simulink model "IEEE33_TR_TEMPORAL_RECOGNIZABILITY_MASTER"  (R2026b)
settings: Solver=ode23t  StopTime=0.2  MaxStep=1e-5
undefined symbols (not defined in the file): Three_PhaseBreaker_class, Three_PhaseSeriesRLCLoad_class, Three_PhaseSource_class, Three_PhaseV_IMeasuremen_class
libraries: ee_lib x146, nesl_utility x106, fl_lib x33, eeRmsMeasurement x2
(part 6 of 7)

== system IEEE33_TR_TEMPORAL_RECOGNIZABILITY_MASTER/Bus_3/CB3-1 ==
  com : Inport
  Add : Sum
  Circuit Breaker : ee_lib/Switches & Breakers/Circuit Breaker (Three-Phase)  port_option=ee.enum.threePhasePort.expanded  control_port_option=ee.enum.controlport.ps  R_closed=0.01 Ohm  G_open=Three_PhaseBreaker_class('open',1000000,Inf,[0.0166666666666667 0.0833333333333333],'on').objParamMappingDerived.NewDerivedParam.G_open 1/Ohm  threshold=0.5 V  breaker_behavior=ee.enum.switches.breakerBehavior.zeroCrossingEnable  i_th=1e-8 A
  Data Type Conversion : DataTypeConversion  OutDataTypeStr=double  SaturateOnIntegerOverflow=off  RndMeth=Floor
  NOT : Logic  Operator=NOT  IconShape=distinctive  AllPortsSameDT=off  OutDataTypeStr=boolean
  Simulink-PS Converter : nesl_utility/Simulink-PS Converter  PhysicalDomain=network_engine_domain  SubClassName=ps_input  LeftPortType=input  RightPortType=output  PseudoPeriodic=off  Frequencies=[]  NoiseDistribution=none  NoiseParameters=[]  Unit=1  AffineConversion=off  FilteringAndDerivatives=provide  SimscapeFilterOrder=1  InputFilterTimeConstant=0.001  UdotUserProvided=0
  Step : Step  Time=1e-6  InitialValue=Three_PhaseBreaker_class('open',1000000,Inf,[0.0166666666666667 0.0833333333333333],'on').objParamMappingDerived.NewDerivedParam.StepInitialValue  FinalValue=0  SampleTime=0
  A : PMIOPort  Side=Left
  B : PMIOPort  Port=2  Side=Left
  C : PMIOPort  Port=3  Side=Left
  a : PMIOPort  Port=4  Side=Right
  b : PMIOPort  Port=5  Side=Right
  c : PMIOPort  Port=6  Side=Right
  wires:
  com/1 -> Add/1
  Add/1 -> NOT/1
  Step/1 -> Add/2
  Data Type Conversion/1 -> Simulink-PS Converter/1
  NOT/1 -> Data Type Conversion/1
  connections:
  Circuit Breaker/LConn1 -- Simulink-PS Converter/RConn1
  c/RConn1 -- Circuit Breaker/RConn3
  b/RConn1 -- Circuit Breaker/RConn2
  a/RConn1 -- Circuit Breaker/RConn1
  Circuit Breaker/LConn4 -- C/RConn1
  Circuit Breaker/LConn3 -- B/RConn1
  Circuit Breaker/LConn2 -- A/RConn1

== system IEEE33_TR_TEMPORAL_RECOGNIZABILITY_MASTER/Bus_3/CB3-2 ==
  com : Inport
  Add : Sum
  Circuit Breaker : ee_lib/Switches & Breakers/Circuit Breaker (Three-Phase)  port_option=ee.enum.threePhasePort.expanded  control_port_option=ee.enum.controlport.ps  R_closed=0.01 Ohm  G_open=Three_PhaseBreaker_class('open',1000000,Inf,[0.0166666666666667 0.0833333333333333],'on').objParamMappingDerived.NewDerivedParam.G_open 1/Ohm  threshold=0.5 V  breaker_behavior=ee.enum.switches.breakerBehavior.zeroCrossingEnable  i_th=1e-8 A
  Data Type Conversion : DataTypeConversion  OutDataTypeStr=double  SaturateOnIntegerOverflow=off  RndMeth=Floor
  NOT : Logic  Operator=NOT  IconShape=distinctive  AllPortsSameDT=off  OutDataTypeStr=boolean
  Simulink-PS Converter : nesl_utility/Simulink-PS Converter  PhysicalDomain=network_engine_domain  SubClassName=ps_input  LeftPortType=input  RightPortType=output  PseudoPeriodic=off  Frequencies=[]  NoiseDistribution=none  NoiseParameters=[]  Unit=1  AffineConversion=off  FilteringAndDerivatives=provide  SimscapeFilterOrder=1  InputFilterTimeConstant=0.001  UdotUserProvided=0
  Step : Step  Time=1e-6  InitialValue=Three_PhaseBreaker_class('open',1000000,Inf,[0.0166666666666667 0.0833333333333333],'on').objParamMappingDerived.NewDerivedParam.StepInitialValue  FinalValue=0  SampleTime=0
  A : PMIOPort  Side=Left
  B : PMIOPort  Port=2  Side=Left
  C : PMIOPort  Port=3  Side=Left
  a : PMIOPort  Port=4  Side=Right
  b : PMIOPort  Port=5  Side=Right
  c : PMIOPort  Port=6  Side=Right
  wires:
  com/1 -> Add/1
  Add/1 -> NOT/1
  Step/1 -> Add/2
  Data Type Conversion/1 -> Simulink-PS Converter/1
  NOT/1 -> Data Type Conversion/1
  connections:
  Circuit Breaker/LConn1 -- Simulink-PS Converter/RConn1
  c/RConn1 -- Circuit Breaker/RConn3
  b/RConn1 -- Circuit Breaker/RConn2
  a/RConn1 -- Circuit Breaker/RConn1
  Circuit Breaker/LConn4 -- C/RConn1
  Circuit Breaker/LConn3 -- B/RConn1
  Circuit Breaker/LConn2 -- A/RConn1

== system IEEE33_TR_TEMPORAL_RECOGNIZABILITY_MASTER/Bus_3/VI Recorder6 ==
  Vrec : Inport
  Irec : Inport  Port=2
  tag scope: I2to3=global, V2to3=global
  wires:
  Vrec/1 -> [V2to3]
  Irec/1 -> [I2to3]

== system IEEE33_TR_TEMPORAL_RECOGNIZABILITY_MASTER/Bus_30/Bus Load 30 ==
  Electrical Reference : fl_lib/Electrical/Electrical Elements/Electrical Reference
  Wye-Connected Load : ee_lib/Passive/RLC Assemblies/Wye-Connected Load  port_option=ee.enum.threePhasePort.expanded  parameterization=2  component_structure=4  component_structure_PQ=4  R=1 Ohm  L=0.001 H  C=1e-6 F  VRated=11673.3176 V  FRated=60 Hz  P=200000 W  Qpos=600000 V*A  Qneg=Three_PhaseSeriesRLCLoad_class(0).objParamMappingDerived.NewDerivedParam.Qneg V*A  R_parasitic=1e-6 Ohm  G_parasitic=1e-6 1/Ohm  R_parasitic_PQ=1e-6 Ohm  G_parasitic_PQ=1e-6 1/Ohm  Vmag0=11673.3176 V  Vang0=0 deg  Freq0=60 Hz  IL_specify=on  IL_priority=High  IL=[ 0 0 0 ] A  IL_nominal_specify=off  IL_nominal_value=1  IL_nominal_unit=A  VC_specify=on  VC_priority=High  VC=[ 0 0 0 ] V  VC_nominal_specify=off  VC_nominal_value=1  VC_nominal_unit=V
  A : PMIOPort  Side=Left
  B : PMIOPort  Port=2  Side=Left
  C : PMIOPort  Port=3  Side=Left
  connections:
  Electrical Reference/LConn1 -- Wye-Connected Load/RConn1
  Wye-Connected Load/LConn3 -- C/RConn1
  Wye-Connected Load/LConn1 -- A/RConn1
  Wye-Connected Load/LConn2 -- B/RConn1

== system IEEE33_TR_TEMPORAL_RECOGNIZABILITY_MASTER/Bus_30/Bus_30 ==
  Current and Voltage Sensor (Three-Phase) : ee_lib/Sensors & Transducers/Current and Voltage Sensor (Three-Phase)  port_option=ee.enum.threePhasePort.expanded  vMeasurementType=1  outputUnit=2  SRated=100000000 V*A  VRated=500000 V  I_specify=off  I_priority=None  I=[ 0 0 0 ] A  I_nominal_specify=off  I_nominal_value=1  I_nominal_unit=A  V_specify=off  V_priority=None  V=[ 0 0 0 ] V  V_nominal_specify=off  V_nominal_value=1  V_nominal_unit=V
  Igain : Gain  Gain=Three_PhaseV_IMeasuremen_class('phase-to-phase','yes','off','off','off',100000000,500000).objParamMappingDerived.NewDerivedParam.IG
  PS-Simulink Converter : nesl_utility/PS-Simulink Converter  PhysicalDomain=network_engine_domain  SubClassName=ps_output  LeftPortType=input  RightPortType=output  PseudoPeriodic=off  Frequencies=[]  VectorFormat=1-D array  Unit=1  AffineConversion=off
  PS-Simulink Converter1 : nesl_utility/PS-Simulink Converter  PhysicalDomain=network_engine_domain  SubClassName=ps_output  LeftPortType=input  RightPortType=output  PseudoPeriodic=off  Frequencies=[]  VectorFormat=1-D array  Unit=1  AffineConversion=off
  Vgain : Gain  Gain=Three_PhaseV_IMeasuremen_class('phase-to-phase','yes','off','off','off',100000000,500000).objParamMappingDerived.NewDerivedParam.VG
  A : PMIOPort  Side=Left
  B : PMIOPort  Port=2  Side=Left
  C : PMIOPort  Port=3  Side=Left
  a : PMIOPort  Port=4  Side=Right
  b : PMIOPort  Port=5  Side=Right
  c : PMIOPort  Port=6  Side=Right
  Vabc : Outport  VectorParamsAs1DForOutWhenUnconnected=off
  Iabc : Outport  Port=2  VectorParamsAs1DForOutWhenUnconnected=off
  wires:
  Igain/1 -> Iabc/1
  Vgain/1 -> Vabc/1
  PS-Simulink Converter1/1 -> Igain/1
  PS-Simulink Converter/1 -> Vgain/1
  connections:
  Current and Voltage Sensor (Three-Phase)/RConn1 -- PS-Simulink Converter/LConn1
  Current and Voltage Sensor (Three-Phase)/RConn2 -- PS-Simulink Converter1/LConn1
  Current and Voltage Sensor (Three-Phase)/RConn5 -- c/RConn1
  Current and Voltage Sensor (Three-Phase)/RConn4 -- b/RConn1
  Current and Voltage Sensor (Three-Phase)/RConn3 -- a/RConn1
  Current and Voltage Sensor (Three-Phase)/LConn3 -- C/RConn1
  Current and Voltage Sensor (Three-Phase)/LConn1 -- A/RConn1
  Current and Voltage Sensor (Three-Phase)/LConn2 -- B/RConn1

== system IEEE33_TR_TEMPORAL_RECOGNIZABILITY_MASTER/Bus_30/CB3-2 ==
  com : Inport
  Add : Sum
  Circuit Breaker : ee_lib/Switches & Breakers/Circuit Breaker (Three-Phase)  port_option=ee.enum.threePhasePort.expanded  control_port_option=ee.enum.controlport.ps  R_closed=0.01 Ohm  G_open=Three_PhaseBreaker_class('open',1000000,Inf,[0.0166666666666667 0.0833333333333333],'on').objParamMappingDerived.NewDerivedParam.G_open 1/Ohm  threshold=0.5 V  breaker_behavior=ee.enum.switches.breakerBehavior.zeroCrossingEnable  i_th=1e-8 A
  Data Type Conversion : DataTypeConversion  OutDataTypeStr=double  SaturateOnIntegerOverflow=off  RndMeth=Floor
  NOT : Logic  Operator=NOT  IconShape=distinctive  AllPortsSameDT=off  OutDataTypeStr=boolean
  Simulink-PS Converter : nesl_utility/Simulink-PS Converter  PhysicalDomain=network_engine_domain  SubClassName=ps_input  LeftPortType=input  RightPortType=output  PseudoPeriodic=off  Frequencies=[]  NoiseDistribution=none  NoiseParameters=[]  Unit=1  AffineConversion=off  FilteringAndDerivatives=provide  SimscapeFilterOrder=1  InputFilterTimeConstant=0.001  UdotUserProvided=0
  Step : Step  Time=1e-6  InitialValue=Three_PhaseBreaker_class('open',1000000,Inf,[0.0166666666666667 0.0833333333333333],'on').objParamMappingDerived.NewDerivedParam.StepInitialValue  FinalValue=0  SampleTime=0
  A : PMIOPort  Side=Left
  B : PMIOPort  Port=2  Side=Left
  C : PMIOPort  Port=3  Side=Left
  a : PMIOPort  Port=4  Side=Right
  b : PMIOPort  Port=5  Side=Right
  c : PMIOPort  Port=6  Side=Right
  wires:
  com/1 -> Add/1
  Add/1 -> NOT/1
  Step/1 -> Add/2
  Data Type Conversion/1 -> Simulink-PS Converter/1
  NOT/1 -> Data Type Conversion/1
  connections:
  Circuit Breaker/LConn1 -- Simulink-PS Converter/RConn1
  c/RConn1 -- Circuit Breaker/RConn3
  b/RConn1 -- Circuit Breaker/RConn2
  a/RConn1 -- Circuit Breaker/RConn1
  Circuit Breaker/LConn4 -- C/RConn1
  Circuit Breaker/LConn3 -- B/RConn1
  Circuit Breaker/LConn2 -- A/RConn1

== system IEEE33_TR_TEMPORAL_RECOGNIZABILITY_MASTER/Bus_30/VI Recorder26 ==
  Vrec : Inport
  Irec : Inport  Port=2
  tag scope: I29to30=global, V29to30=global
  wires:
  Vrec/1 -> [V29to30]
  Irec/1 -> [I29to30]

== system IEEE33_TR_TEMPORAL_RECOGNIZABILITY_MASTER/Bus_31/Bus Load 31 ==
  Electrical Reference : fl_lib/Electrical/Electrical Elements/Electrical Reference
  Wye-Connected Load : ee_lib/Passive/RLC Assemblies/Wye-Connected Load  port_option=ee.enum.threePhasePort.expanded  parameterization=2  component_structure=4  component_structure_PQ=4  R=1 Ohm  L=0.001 H  C=1e-6 F  VRated=11620.7279 V  FRated=60 Hz  P=150000 W  Qpos=70000 V*A  Qneg=Three_PhaseSeriesRLCLoad_class(0).objParamMappingDerived.NewDerivedParam.Qneg V*A  R_parasitic=1e-6 Ohm  G_parasitic=1e-6 1/Ohm  R_parasitic_PQ=1e-6 Ohm  G_parasitic_PQ=1e-6 1/Ohm  Vmag0=11620.7279 V  Vang0=0 deg  Freq0=60 Hz  IL_specify=on  IL_priority=High  IL=[ 0 0 0 ] A  IL_nominal_specify=off  IL_nominal_value=1  IL_nominal_unit=A  VC_specify=on  VC_priority=High  VC=[ 0 0 0 ] V  VC_nominal_specify=off  VC_nominal_value=1  VC_nominal_unit=V
  A : PMIOPort  Side=Left
  B : PMIOPort  Port=2  Side=Left
  C : PMIOPort  Port=3  Side=Left
  connections:
  Electrical Reference/LConn1 -- Wye-Connected Load/RConn1
  Wye-Connected Load/LConn3 -- C/RConn1
  Wye-Connected Load/LConn1 -- A/RConn1
  Wye-Connected Load/LConn2 -- B/RConn1

== system IEEE33_TR_TEMPORAL_RECOGNIZABILITY_MASTER/Bus_31/Bus_31 ==
  Current and Voltage Sensor (Three-Phase) : ee_lib/Sensors & Transducers/Current and Voltage Sensor (Three-Phase)  port_option=ee.enum.threePhasePort.expanded  vMeasurementType=1  outputUnit=2  SRated=100000000 V*A  VRated=500000 V  I_specify=off  I_priority=None  I=[ 0 0 0 ] A  I_nominal_specify=off  I_nominal_value=1  I_nominal_unit=A  V_specify=off  V_priority=None  V=[ 0 0 0 ] V  V_nominal_specify=off  V_nominal_value=1  V_nominal_unit=V
  Igain : Gain  Gain=Three_PhaseV_IMeasuremen_class('phase-to-phase','yes','off','off','off',100000000,500000).objParamMappingDerived.NewDerivedParam.IG
  PS-Simulink Converter : nesl_utility/PS-Simulink Converter  PhysicalDomain=network_engine_domain  SubClassName=ps_output  LeftPortType=input  RightPortType=output  PseudoPeriodic=off  Frequencies=[]  VectorFormat=1-D array  Unit=1  AffineConversion=off
  PS-Simulink Converter1 : nesl_utility/PS-Simulink Converter  PhysicalDomain=network_engine_domain  SubClassName=ps_output  LeftPortType=input  RightPortType=output  PseudoPeriodic=off  Frequencies=[]  VectorFormat=1-D array  Unit=1  AffineConversion=off
  Vgain : Gain  Gain=Three_PhaseV_IMeasuremen_class('phase-to-phase','yes','off','off','off',100000000,500000).objParamMappingDerived.NewDerivedParam.VG
  A : PMIOPort  Side=Left
  B : PMIOPort  Port=2  Side=Left
  C : PMIOPort  Port=3  Side=Left
  a : PMIOPort  Port=4  Side=Right
  b : PMIOPort  Port=5  Side=Right
  c : PMIOPort  Port=6  Side=Right
  Vabc : Outport  VectorParamsAs1DForOutWhenUnconnected=off
  Iabc : Outport  Port=2  VectorParamsAs1DForOutWhenUnconnected=off
  wires:
  Igain/1 -> Iabc/1
  Vgain/1 -> Vabc/1
  PS-Simulink Converter1/1 -> Igain/1
  PS-Simulink Converter/1 -> Vgain/1
  connections:
  Current and Voltage Sensor (Three-Phase)/RConn1 -- PS-Simulink Converter/LConn1
  Current and Voltage Sensor (Three-Phase)/RConn2 -- PS-Simulink Converter1/LConn1
  Current and Voltage Sensor (Three-Phase)/RConn5 -- c/RConn1
  Current and Voltage Sensor (Three-Phase)/RConn4 -- b/RConn1
  Current and Voltage Sensor (Three-Phase)/RConn3 -- a/RConn1
  Current and Voltage Sensor (Three-Phase)/LConn3 -- C/RConn1
  Current and Voltage Sensor (Three-Phase)/LConn1 -- A/RConn1
  Current and Voltage Sensor (Three-Phase)/LConn2 -- B/RConn1

== system IEEE33_TR_TEMPORAL_RECOGNIZABILITY_MASTER/Bus_31/CB3-2 ==
  com : Inport
  Add : Sum
  Circuit Breaker : ee_lib/Switches & Breakers/Circuit Breaker (Three-Phase)  port_option=ee.enum.threePhasePort.expanded  control_port_option=ee.enum.controlport.ps  R_closed=0.01 Ohm  G_open=Three_PhaseBreaker_class('open',1000000,Inf,[0.0166666666666667 0.0833333333333333],'on').objParamMappingDerived.NewDerivedParam.G_open 1/Ohm  threshold=0.5 V  breaker_behavior=ee.enum.switches.breakerBehavior.zeroCrossingEnable  i_th=1e-8 A
  Data Type Conversion : DataTypeConversion  OutDataTypeStr=double  SaturateOnIntegerOverflow=off  RndMeth=Floor
  NOT : Logic  Operator=NOT  IconShape=distinctive  AllPortsSameDT=off  OutDataTypeStr=boolean
  Simulink-PS Converter : nesl_utility/Simulink-PS Converter  PhysicalDomain=network_engine_domain  SubClassName=ps_input  LeftPortType=input  RightPortType=output  PseudoPeriodic=off  Frequencies=[]  NoiseDistribution=none  NoiseParameters=[]  Unit=1  AffineConversion=off  FilteringAndDerivatives=provide  SimscapeFilterOrder=1  InputFilterTimeConstant=0.001  UdotUserProvided=0
  Step : Step  Time=1e-6  InitialValue=Three_PhaseBreaker_class('open',1000000,Inf,[0.0166666666666667 0.0833333333333333],'on').objParamMappingDerived.NewDerivedParam.StepInitialValue  FinalValue=0  SampleTime=0
  A : PMIOPort  Side=Left
  B : PMIOPort  Port=2  Side=Left
  C : PMIOPort  Port=3  Side=Left
  a : PMIOPort  Port=4  Side=Right
  b : PMIOPort  Port=5  Side=Right
  c : PMIOPort  Port=6  Side=Right
  wires:
  com/1 -> Add/1
  Add/1 -> NOT/1
  Step/1 -> Add/2
  Data Type Conversion/1 -> Simulink-PS Converter/1
  NOT/1 -> Data Type Conversion/1
  connections:
  Circuit Breaker/LConn1 -- Simulink-PS Converter/RConn1
  c/RConn1 -- Circuit Breaker/RConn3
  b/RConn1 -- Circuit Breaker/RConn2
  a/RConn1 -- Circuit Breaker/RConn1
  Circuit Breaker/LConn4 -- C/RConn1
  Circuit Breaker/LConn3 -- B/RConn1
  Circuit Breaker/LConn2 -- A/RConn1

== system IEEE33_TR_TEMPORAL_RECOGNIZABILITY_MASTER/Bus_31/VI Recorder27 ==
  Vrec : Inport
  Irec : Inport  Port=2
  tag scope: I30to31=global, V30to31=global
  wires:
  Vrec/1 -> [V30to31]
  Irec/1 -> [I30to31]

== system IEEE33_TR_TEMPORAL_RECOGNIZABILITY_MASTER/Bus_32/Bus Load 32 ==
  Electrical Reference : fl_lib/Electrical/Electrical Elements/Electrical Reference
  Wye-Connected Load : ee_lib/Passive/RLC Assemblies/Wye-Connected Load  port_option=ee.enum.threePhasePort.expanded  parameterization=2  component_structure=4  component_structure_PQ=4  R=1 Ohm  L=0.001 H  C=1e-6 F  VRated=11609.1567 V  FRated=60 Hz  P=210000 W  Qpos=100000 V*A  Qneg=Three_PhaseSeriesRLCLoad_class(0).objParamMappingDerived.NewDerivedParam.Qneg V*A  R_parasitic=1e-6 Ohm  G_parasitic=1e-6 1/Ohm  R_parasitic_PQ=1e-6 Ohm  G_parasitic_PQ=1e-6 1/Ohm  Vmag0=11609.1567 V  Vang0=0 deg  Freq0=60 Hz  IL_specify=on  IL_priority=High  IL=[ 0 0 0 ] A  IL_nominal_specify=off  IL_nominal_value=1  IL_nominal_unit=A  VC_specify=on  VC_priority=High  VC=[ 0 0 0 ] V  VC_nominal_specify=off  VC_nominal_value=1  VC_nominal_unit=V
  A : PMIOPort  Side=Left
  B : PMIOPort  Port=2  Side=Left
  C : PMIOPort  Port=3  Side=Left
  connections:
  Electrical Reference/LConn1 -- Wye-Connected Load/RConn1
  Wye-Connected Load/LConn3 -- C/RConn1
  Wye-Connected Load/LConn1 -- A/RConn1
  Wye-Connected Load/LConn2 -- B/RConn1

== system IEEE33_TR_TEMPORAL_RECOGNIZABILITY_MASTER/Bus_32/Bus_32 ==
  Current and Voltage Sensor (Three-Phase) : ee_lib/Sensors & Transducers/Current and Voltage Sensor (Three-Phase)  port_option=ee.enum.threePhasePort.expanded  vMeasurementType=1  outputUnit=2  SRated=100000000 V*A  VRated=500000 V  I_specify=off  I_priority=None  I=[ 0 0 0 ] A  I_nominal_specify=off  I_nominal_value=1  I_nominal_unit=A  V_specify=off  V_priority=None  V=[ 0 0 0 ] V  V_nominal_specify=off  V_nominal_value=1  V_nominal_unit=V
  Igain : Gain  Gain=Three_PhaseV_IMeasuremen_class('phase-to-phase','yes','off','off','off',100000000,500000).objParamMappingDerived.NewDerivedParam.IG
  PS-Simulink Converter : nesl_utility/PS-Simulink Converter  PhysicalDomain=network_engine_domain  SubClassName=ps_output  LeftPortType=input  RightPortType=output  PseudoPeriodic=off  Frequencies=[]  VectorFormat=1-D array  Unit=1  AffineConversion=off
  PS-Simulink Converter1 : nesl_utility/PS-Simulink Converter  PhysicalDomain=network_engine_domain  SubClassName=ps_output  LeftPortType=input  RightPortType=output  PseudoPeriodic=off  Frequencies=[]  VectorFormat=1-D array  Unit=1  AffineConversion=off
  Vgain : Gain  Gain=Three_PhaseV_IMeasuremen_class('phase-to-phase','yes','off','off','off',100000000,500000).objParamMappingDerived.NewDerivedParam.VG
  A : PMIOPort  Side=Left
  B : PMIOPort  Port=2  Side=Left
  C : PMIOPort  Port=3  Side=Left
  a : PMIOPort  Port=4  Side=Right
  b : PMIOPort  Port=5  Side=Right
  c : PMIOPort  Port=6  Side=Right
  Vabc : Outport  VectorParamsAs1DForOutWhenUnconnected=off
  Iabc : Outport  Port=2  VectorParamsAs1DForOutWhenUnconnected=off
  wires:
  Igain/1 -> Iabc/1
  Vgain/1 -> Vabc/1
  PS-Simulink Converter1/1 -> Igain/1
  PS-Simulink Converter/1 -> Vgain/1
  connections:
  Current and Voltage Sensor (Three-Phase)/RConn1 -- PS-Simulink Converter/LConn1
  Current and Voltage Sensor (Three-Phase)/RConn2 -- PS-Simulink Converter1/LConn1
  Current and Voltage Sensor (Three-Phase)/RConn5 -- c/RConn1
  Current and Voltage Sensor (Three-Phase)/RConn4 -- b/RConn1
  Current and Voltage Sensor (Three-Phase)/RConn3 -- a/RConn1
  Current and Voltage Sensor (Three-Phase)/LConn3 -- C/RConn1
  Current and Voltage Sensor (Three-Phase)/LConn1 -- A/RConn1
  Current and Voltage Sensor (Three-Phase)/LConn2 -- B/RConn1

== system IEEE33_TR_TEMPORAL_RECOGNIZABILITY_MASTER/Bus_32/CB3-2 ==
  com : Inport
  Add : Sum
  Circuit Breaker : ee_lib/Switches & Breakers/Circuit Breaker (Three-Phase)  port_option=ee.enum.threePhasePort.expanded  control_port_option=ee.enum.controlport.ps  R_closed=0.01 Ohm  G_open=Three_PhaseBreaker_class('open',1000000,Inf,[0.0166666666666667 0.0833333333333333],'on').objParamMappingDerived.NewDerivedParam.G_open 1/Ohm  threshold=0.5 V  breaker_behavior=ee.enum.switches.breakerBehavior.zeroCrossingEnable  i_th=1e-8 A
  Data Type Conversion : DataTypeConversion  OutDataTypeStr=double  SaturateOnIntegerOverflow=off  RndMeth=Floor
  NOT : Logic  Operator=NOT  IconShape=distinctive  AllPortsSameDT=off  OutDataTypeStr=boolean
  Simulink-PS Converter : nesl_utility/Simulink-PS Converter  PhysicalDomain=network_engine_domain  SubClassName=ps_input  LeftPortType=input  RightPortType=output  PseudoPeriodic=off  Frequencies=[]  NoiseDistribution=none  NoiseParameters=[]  Unit=1  AffineConversion=off  FilteringAndDerivatives=provide  SimscapeFilterOrder=1  InputFilterTimeConstant=0.001  UdotUserProvided=0
  Step : Step  Time=1e-6  InitialValue=Three_PhaseBreaker_class('open',1000000,Inf,[0.0166666666666667 0.0833333333333333],'on').objParamMappingDerived.NewDerivedParam.StepInitialValue  FinalValue=0  SampleTime=0
  A : PMIOPort  Side=Left
  B : PMIOPort  Port=2  Side=Left
  C : PMIOPort  Port=3  Side=Left
  a : PMIOPort  Port=4  Side=Right
  b : PMIOPort  Port=5  Side=Right
  c : PMIOPort  Port=6  Side=Right
  wires:
  com/1 -> Add/1
  Add/1 -> NOT/1
  Step/1 -> Add/2
  Data Type Conversion/1 -> Simulink-PS Converter/1
  NOT/1 -> Data Type Conversion/1
  connections:
  Circuit Breaker/LConn1 -- Simulink-PS Converter/RConn1
  c/RConn1 -- Circuit Breaker/RConn3
  b/RConn1 -- Circuit Breaker/RConn2
  a/RConn1 -- Circuit Breaker/RConn1
  Circuit Breaker/LConn4 -- C/RConn1
  Circuit Breaker/LConn3 -- B/RConn1
  Circuit Breaker/LConn2 -- A/RConn1

== system IEEE33_TR_TEMPORAL_RECOGNIZABILITY_MASTER/Bus_32/VI Recorder28 ==
  Vrec : Inport
  Irec : Inport  Port=2
  tag scope: I31to32=global, V31to32=global
  wires:
  Vrec/1 -> [V31to32]
  Irec/1 -> [I31to32]

== system IEEE33_TR_TEMPORAL_RECOGNIZABILITY_MASTER/Bus_33/Bus Load 33 ==
  Electrical Reference : fl_lib/Electrical/Electrical Elements/Electrical Reference
  Wye-Connected Load : ee_lib/Passive/RLC Assemblies/Wye-Connected Load  port_option=ee.enum.threePhasePort.expanded  parameterization=2  component_structure=4  component_structure_PQ=4  R=1 Ohm  L=0.001 H  C=1e-6 F  VRated=11605.5739 V  FRated=60 Hz  P=60000 W  Qpos=40000 V*A  Qneg=Three_PhaseSeriesRLCLoad_class(0).objParamMappingDerived.NewDerivedParam.Qneg V*A  R_parasitic=1e-6 Ohm  G_parasitic=1e-6 1/Ohm  R_parasitic_PQ=1e-6 Ohm  G_parasitic_PQ=1e-6 1/Ohm  Vmag0=11605.5739 V  Vang0=0 deg  Freq0=60 Hz  IL_specify=on  IL_priority=High  IL=[ 0 0 0 ] A  IL_nominal_specify=off  IL_nominal_value=1  IL_nominal_unit=A  VC_specify=on  VC_priority=High  VC=[ 0 0 0 ] V  VC_nominal_specify=off  VC_nominal_value=1  VC_nominal_unit=V
  A : PMIOPort  Side=Left
  B : PMIOPort  Port=2  Side=Left
  C : PMIOPort  Port=3  Side=Left
  connections:
  Electrical Reference/LConn1 -- Wye-Connected Load/RConn1
  Wye-Connected Load/LConn3 -- C/RConn1
  Wye-Connected Load/LConn1 -- A/RConn1
  Wye-Connected Load/LConn2 -- B/RConn1

== system IEEE33_TR_TEMPORAL_RECOGNIZABILITY_MASTER/Bus_33/Bus_33 ==
  Current and Voltage Sensor (Three-Phase) : ee_lib/Sensors & Transducers/Current and Voltage Sensor (Three-Phase)  port_option=ee.enum.threePhasePort.expanded  vMeasurementType=1  outputUnit=2  SRated=100000000 V*A  VRated=500000 V  I_specify=off  I_priority=None  I=[ 0 0 0 ] A  I_nominal_specify=off  I_nominal_value=1  I_nominal_unit=A  V_specify=off  V_priority=None  V=[ 0 0 0 ] V  V_nominal_specify=off  V_nominal_value=1  V_nominal_unit=V
  Igain : Gain  Gain=Three_PhaseV_IMeasuremen_class('phase-to-phase','yes','off','off','off',100000000,500000).objParamMappingDerived.NewDerivedParam.IG
  PS-Simulink Converter : nesl_utility/PS-Simulink Converter  PhysicalDomain=network_engine_domain  SubClassName=ps_output  LeftPortType=input  RightPortType=output  PseudoPeriodic=off  Frequencies=[]  VectorFormat=1-D array  Unit=1  AffineConversion=off
  PS-Simulink Converter1 : nesl_utility/PS-Simulink Converter  PhysicalDomain=network_engine_domain  SubClassName=ps_output  LeftPortType=input  RightPortType=output  PseudoPeriodic=off  Frequencies=[]  VectorFormat=1-D array  Unit=1  AffineConversion=off
  Vgain : Gain  Gain=Three_PhaseV_IMeasuremen_class('phase-to-phase','yes','off','off','off',100000000,500000).objParamMappingDerived.NewDerivedParam.VG
  A : PMIOPort  Side=Left
  B : PMIOPort  Port=2  Side=Left
  C : PMIOPort  Port=3  Side=Left
  a : PMIOPort  Port=4  Side=Right
  b : PMIOPort  Port=5  Side=Right
  c : PMIOPort  Port=6  Side=Right
  Vabc : Outport  VectorParamsAs1DForOutWhenUnconnected=off
  Iabc : Outport  Port=2  VectorParamsAs1DForOutWhenUnconnected=off
  wires:
  Igain/1 -> Iabc/1
  Vgain/1 -> Vabc/1
  PS-Simulink Converter1/1 -> Igain/1
  PS-Simulink Converter/1 -> Vgain/1
  connections:
  Current and Voltage Sensor (Three-Phase)/RConn1 -- PS-Simulink Converter/LConn1
  Current and Voltage Sensor (Three-Phase)/RConn2 -- PS-Simulink Converter1/LConn1
  Current and Voltage Sensor (Three-Phase)/RConn5 -- c/RConn1
  Current and Voltage Sensor (Three-Phase)/RConn4 -- b/RConn1
  Current and Voltage Sensor (Three-Phase)/RConn3 -- a/RConn1
  Current and Voltage Sensor (Three-Phase)/LConn3 -- C/RConn1
  Current and Voltage Sensor (Three-Phase)/LConn1 -- A/RConn1
  Current and Voltage Sensor (Three-Phase)/LConn2 -- B/RConn1

== system IEEE33_TR_TEMPORAL_RECOGNIZABILITY_MASTER/Bus_33/VI Recorder29 ==
  Vrec : Inport
  Irec : Inport  Port=2
  tag scope: I32to33=global, V32to33=global
  wires:
  Vrec/1 -> [V32to33]
  Irec/1 -> [I32to33]

== system IEEE33_TR_TEMPORAL_RECOGNIZABILITY_MASTER/Bus_4/Bus Load 4 ==
  Electrical Reference : fl_lib/Electrical/Electrical Elements/Electrical Reference
  Wye-Connected Load : ee_lib/Passive/RLC Assemblies/Wye-Connected Load  port_option=ee.enum.threePhasePort.expanded  parameterization=2  component_structure=4  component_structure_PQ=4  R=1 Ohm  L=0.001 H  C=1e-6 F  VRated=12349.6274 V  FRated=60 Hz  P=120000 W  Qpos=80000 V*A  Qneg=Three_PhaseSeriesRLCLoad_class(0).objParamMappingDerived.NewDerivedParam.Qneg V*A  R_parasitic=1e-6 Ohm  G_parasitic=1e-6 1/Ohm  R_parasitic_PQ=1e-6 Ohm  G_parasitic_PQ=1e-6 1/Ohm  Vmag0=12349.6274 V  Vang0=0 deg  Freq0=60 Hz  IL_specify=on  IL_priority=High  IL=[ 0 0 0 ] A  IL_nominal_specify=off  IL_nominal_value=1  IL_nominal_unit=A  VC_specify=on  VC_priority=High  VC=[ 0 0 0 ] V  VC_nominal_specify=off  VC_nominal_value=1  VC_nominal_unit=V
  A : PMIOPort  Side=Left
  B : PMIOPort  Port=2  Side=Left
  C : PMIOPort  Port=3  Side=Left
  connections:
  Electrical Reference/LConn1 -- Wye-Connected Load/RConn1
  Wye-Connected Load/LConn3 -- C/RConn1
  Wye-Connected Load/LConn1 -- A/RConn1
  Wye-Connected Load/LConn2 -- B/RConn1

== system IEEE33_TR_TEMPORAL_RECOGNIZABILITY_MASTER/Bus_4/Bus_4 ==
  Current and Voltage Sensor (Three-Phase) : ee_lib/Sensors & Transducers/Current and Voltage Sensor (Three-Phase)  port_option=ee.enum.threePhasePort.expanded  vMeasurementType=1  outputUnit=2  SRated=100000000 V*A  VRated=500000 V  I_specify=off  I_priority=None  I=[ 0 0 0 ] A  I_nominal_specify=off  I_nominal_value=1  I_nominal_unit=A  V_specify=off  V_priority=None  V=[ 0 0 0 ] V  V_nominal_specify=off  V_nominal_value=1  V_nominal_unit=V
  Igain : Gain  Gain=Three_PhaseV_IMeasuremen_class('phase-to-phase','yes','off','off','off',100000000,500000).objParamMappingDerived.NewDerivedParam.IG
  PS-Simulink Converter : nesl_utility/PS-Simulink Converter  PhysicalDomain=network_engine_domain  SubClassName=ps_output  LeftPortType=input  RightPortType=output  PseudoPeriodic=off  Frequencies=[]  VectorFormat=1-D array  Unit=1  AffineConversion=off
  PS-Simulink Converter1 : nesl_utility/PS-Simulink Converter  PhysicalDomain=network_engine_domain  SubClassName=ps_output  LeftPortType=input  RightPortType=output  PseudoPeriodic=off  Frequencies=[]  VectorFormat=1-D array  Unit=1  AffineConversion=off
  Vgain : Gain  Gain=Three_PhaseV_IMeasuremen_class('phase-to-phase','yes','off','off','off',100000000,500000).objParamMappingDerived.NewDerivedParam.VG
  A : PMIOPort  Side=Left
  B : PMIOPort  Port=2  Side=Left
  C : PMIOPort  Port=3  Side=Left
  a : PMIOPort  Port=4  Side=Right
  b : PMIOPort  Port=5  Side=Right
  c : PMIOPort  Port=6  Side=Right
  Vabc : Outport  VectorParamsAs1DForOutWhenUnconnected=off
  Iabc : Outport  Port=2  VectorParamsAs1DForOutWhenUnconnected=off
  wires:
  Igain/1 -> Iabc/1
  Vgain/1 -> Vabc/1
  PS-Simulink Converter1/1 -> Igain/1
  PS-Simulink Converter/1 -> Vgain/1
  connections:
  Current and Voltage Sensor (Three-Phase)/RConn1 -- PS-Simulink Converter/LConn1
  Current and Voltage Sensor (Three-Phase)/RConn2 -- PS-Simulink Converter1/LConn1
  Current and Voltage Sensor (Three-Phase)/RConn5 -- c/RConn1
  Current and Voltage Sensor (Three-Phase)/RConn4 -- b/RConn1
  Current and Voltage Sensor (Three-Phase)/RConn3 -- a/RConn1
  Current and Voltage Sensor (Three-Phase)/LConn3 -- C/RConn1
  Current and Voltage Sensor (Three-Phase)/LConn1 -- A/RConn1
  Current and Voltage Sensor (Three-Phase)/LConn2 -- B/RConn1

== system IEEE33_TR_TEMPORAL_RECOGNIZABILITY_MASTER/Bus_4/CB3-2 ==
  com : Inport
  Add : Sum
  Circuit Breaker : ee_lib/Switches & Breakers/Circuit Breaker (Three-Phase)  port_option=ee.enum.threePhasePort.expanded  control_port_option=ee.enum.controlport.ps  R_closed=0.01 Ohm  G_open=Three_PhaseBreaker_class('open',1000000,Inf,[0.0166666666666667 0.0833333333333333],'on').objParamMappingDerived.NewDerivedParam.G_open 1/Ohm  threshold=0.5 V  breaker_behavior=ee.enum.switches.breakerBehavior.zeroCrossingEnable  i_th=1e-8 A
  Data Type Conversion : DataTypeConversion  OutDataTypeStr=double  SaturateOnIntegerOverflow=off  RndMeth=Floor
  NOT : Logic  Operator=NOT  IconShape=distinctive  AllPortsSameDT=off  OutDataTypeStr=boolean
  Simulink-PS Converter : nesl_utility/Simulink-PS Converter  PhysicalDomain=network_engine_domain  SubClassName=ps_input  LeftPortType=input  RightPortType=output  PseudoPeriodic=off  Frequencies=[]  NoiseDistribution=none  NoiseParameters=[]  Unit=1  AffineConversion=off  FilteringAndDerivatives=provide  SimscapeFilterOrder=1  InputFilterTimeConstant=0.001  UdotUserProvided=0
  Step : Step  Time=1e-6  InitialValue=Three_PhaseBreaker_class('open',1000000,Inf,[0.0166666666666667 0.0833333333333333],'on').objParamMappingDerived.NewDerivedParam.StepInitialValue  FinalValue=0  SampleTime=0
  A : PMIOPort  Side=Left
  B : PMIOPort  Port=2  Side=Left
  C : PMIOPort  Port=3  Side=Left
  a : PMIOPort  Port=4  Side=Right
  b : PMIOPort  Port=5  Side=Right
  c : PMIOPort  Port=6  Side=Right
  wires:
  com/1 -> Add/1
  Add/1 -> NOT/1
  Step/1 -> Add/2
  Data Type Conversion/1 -> Simulink-PS Converter/1
  NOT/1 -> Data Type Conversion/1
  connections:
  Circuit Breaker/LConn1 -- Simulink-PS Converter/RConn1
  c/RConn1 -- Circuit Breaker/RConn3
  b/RConn1 -- Circuit Breaker/RConn2
  a/RConn1 -- Circuit Breaker/RConn1
  Circuit Breaker/LConn4 -- C/RConn1
  Circuit Breaker/LConn3 -- B/RConn1
  Circuit Breaker/LConn2 -- A/RConn1

== system IEEE33_TR_TEMPORAL_RECOGNIZABILITY_MASTER/Bus_4/VI Recorder7 ==
  Vrec : Inport
  Irec : Inport  Port=2
  tag scope: I3to4=global, V3to4=global
  wires:
  Vrec/1 -> [V3to4]
  Irec/1 -> [I3to4]

== system IEEE33_TR_TEMPORAL_RECOGNIZABILITY_MASTER/Bus_5/Bus Load 5 ==
  Electrical Reference : fl_lib/Electrical/Electrical Elements/Electrical Reference
  Wye-Connected Load : ee_lib/Passive/RLC Assemblies/Wye-Connected Load  port_option=ee.enum.threePhasePort.expanded  parameterization=2  component_structure=4  component_structure_PQ=4  R=1 Ohm  L=0.001 H  C=1e-6 F  VRated=12256.1207 V  FRated=60 Hz  P=60000 W  Qpos=30000 V*A  Qneg=Three_PhaseSeriesRLCLoad_class(0).objParamMappingDerived.NewDerivedParam.Qneg V*A  R_parasitic=1e-6 Ohm  G_parasitic=1e-6 1/Ohm  R_parasitic_PQ=1e-6 Ohm  G_parasitic_PQ=1e-6 1/Ohm  Vmag0=12256.1207 V  Vang0=0 deg  Freq0=60 Hz  IL_specify=on  IL_priority=High  IL=[ 0 0 0 ] A  IL_nominal_specify=off  IL_nominal_value=1  IL_nominal_unit=A  VC_specify=on  VC_priority=High  VC=[ 0 0 0 ] V  VC_nominal_specify=off  VC_nominal_value=1  VC_nominal_unit=V
  A : PMIOPort  Side=Left
  B : PMIOPort  Port=2  Side=Left
  C : PMIOPort  Port=3  Side=Left
  connections:
  Electrical Reference/LConn1 -- Wye-Connected Load/RConn1
  Wye-Connected Load/LConn3 -- C/RConn1
  Wye-Connected Load/LConn1 -- A/RConn1
  Wye-Connected Load/LConn2 -- B/RConn1

== system IEEE33_TR_TEMPORAL_RECOGNIZABILITY_MASTER/Bus_5/Bus_5 ==
  Current and Voltage Sensor (Three-Phase) : ee_lib/Sensors & Transducers/Current and Voltage Sensor (Three-Phase)  port_option=ee.enum.threePhasePort.expanded  vMeasurementType=1  outputUnit=2  SRated=100000000 V*A  VRated=500000 V  I_specify=off  I_priority=None  I=[ 0 0 0 ] A  I_nominal_specify=off  I_nominal_value=1  I_nominal_unit=A  V_specify=off  V_priority=None  V=[ 0 0 0 ] V  V_nominal_specify=off  V_nominal_value=1  V_nominal_unit=V
  Igain : Gain  Gain=Three_PhaseV_IMeasuremen_class('phase-to-phase','yes','off','off','off',100000000,500000).objParamMappingDerived.NewDerivedParam.IG
  PS-Simulink Converter : nesl_utility/PS-Simulink Converter  PhysicalDomain=network_engine_domain  SubClassName=ps_output  LeftPortType=input  RightPortType=output  PseudoPeriodic=off  Frequencies=[]  VectorFormat=1-D array  Unit=1  AffineConversion=off
  PS-Simulink Converter1 : nesl_utility/PS-Simulink Converter  PhysicalDomain=network_engine_domain  SubClassName=ps_output  LeftPortType=input  RightPortType=output  PseudoPeriodic=off  Frequencies=[]  VectorFormat=1-D array  Unit=1  AffineConversion=off
  Vgain : Gain  Gain=Three_PhaseV_IMeasuremen_class('phase-to-phase','yes','off','off','off',100000000,500000).objParamMappingDerived.NewDerivedParam.VG
  A : PMIOPort  Side=Left
  B : PMIOPort  Port=2  Side=Left
  C : PMIOPort  Port=3  Side=Left
  a : PMIOPort  Port=4  Side=Right
  b : PMIOPort  Port=5  Side=Right
  c : PMIOPort  Port=6  Side=Right
  Vabc : Outport  VectorParamsAs1DForOutWhenUnconnected=off
  Iabc : Outport  Port=2  VectorParamsAs1DForOutWhenUnconnected=off
  wires:
  Igain/1 -> Iabc/1
  Vgain/1 -> Vabc/1
  PS-Simulink Converter1/1 -> Igain/1
  PS-Simulink Converter/1 -> Vgain/1
  connections:
  Current and Voltage Sensor (Three-Phase)/RConn1 -- PS-Simulink Converter/LConn1
  Current and Voltage Sensor (Three-Phase)/RConn2 -- PS-Simulink Converter1/LConn1
  Current and Voltage Sensor (Three-Phase)/RConn5 -- c/RConn1
  Current and Voltage Sensor (Three-Phase)/RConn4 -- b/RConn1
  Current and Voltage Sensor (Three-Phase)/RConn3 -- a/RConn1
  Current and Voltage Sensor (Three-Phase)/LConn3 -- C/RConn1
  Current and Voltage Sensor (Three-Phase)/LConn1 -- A/RConn1
  Current and Voltage Sensor (Three-Phase)/LConn2 -- B/RConn1

== system IEEE33_TR_TEMPORAL_RECOGNIZABILITY_MASTER/Bus_5/CB3-2 ==
  com : Inport
  Add : Sum
  Circuit Breaker : ee_lib/Switches & Breakers/Circuit Breaker (Three-Phase)  port_option=ee.enum.threePhasePort.expanded  control_port_option=ee.enum.controlport.ps  R_closed=0.01 Ohm  G_open=Three_PhaseBreaker_class('open',1000000,Inf,[0.0166666666666667 0.0833333333333333],'on').objParamMappingDerived.NewDerivedParam.G_open 1/Ohm  threshold=0.5 V  breaker_behavior=ee.enum.switches.breakerBehavior.zeroCrossingEnable  i_th=1e-8 A
  Data Type Conversion : DataTypeConversion  OutDataTypeStr=double  SaturateOnIntegerOverflow=off  RndMeth=Floor
  NOT : Logic  Operator=NOT  IconShape=distinctive  AllPortsSameDT=off  OutDataTypeStr=boolean
  Simulink-PS Converter : nesl_utility/Simulink-PS Converter  PhysicalDomain=network_engine_domain  SubClassName=ps_input  LeftPortType=input  RightPortType=output  PseudoPeriodic=off  Frequencies=[]  NoiseDistribution=none  NoiseParameters=[]  Unit=1  AffineConversion=off  FilteringAndDerivatives=provide  SimscapeFilterOrder=1  InputFilterTimeConstant=0.001  UdotUserProvided=0
  Step : Step  Time=1e-6  InitialValue=Three_PhaseBreaker_class('open',1000000,Inf,[0.0166666666666667 0.0833333333333333],'on').objParamMappingDerived.NewDerivedParam.StepInitialValue  FinalValue=0  SampleTime=0
  A : PMIOPort  Side=Left
  B : PMIOPort  Port=2  Side=Left
  C : PMIOPort  Port=3  Side=Left
  a : PMIOPort  Port=4  Side=Right
  b : PMIOPort  Port=5  Side=Right
  c : PMIOPort  Port=6  Side=Right
  wires:
  com/1 -> Add/1
  Add/1 -> NOT/1
  Step/1 -> Add/2
  Data Type Conversion/1 -> Simulink-PS Converter/1
  NOT/1 -> Data Type Conversion/1
  connections:
  Circuit Breaker/LConn1 -- Simulink-PS Converter/RConn1
  c/RConn1 -- Circuit Breaker/RConn3
  b/RConn1 -- Circuit Breaker/RConn2
  a/RConn1 -- Circuit Breaker/RConn1
  Circuit Breaker/LConn4 -- C/RConn1
  Circuit Breaker/LConn3 -- B/RConn1
  Circuit Breaker/LConn2 -- A/RConn1

== system IEEE33_TR_TEMPORAL_RECOGNIZABILITY_MASTER/Bus_5/VI Recorder8 ==
  Vrec : Inport
  Irec : Inport  Port=2
  tag scope: I4to5=global, V4to5=global
  wires:
  Vrec/1 -> [V4to5]
  Irec/1 -> [I4to5]

== system IEEE33_TR_TEMPORAL_RECOGNIZABILITY_MASTER/Bus_6/Bus Load 6 ==
  Electrical Reference : fl_lib/Electrical/Electrical Elements/Electrical Reference
  Wye-Connected Load : ee_lib/Passive/RLC Assemblies/Wye-Connected Load  port_option=ee.enum.threePhasePort.expanded  parameterization=2  component_structure=4  component_structure_PQ=4  R=1 Ohm  L=0.001 H  C=1e-6 F  VRated=12023.5058 V  FRated=60 Hz  P=60000 W  Qpos=20000 V*A  Qneg=Three_PhaseSeriesRLCLoad_class(0).objParamMappingDerived.NewDerivedParam.Qneg V*A  R_parasitic=1e-6 Ohm  G_parasitic=1e-6 1/Ohm  R_parasitic_PQ=1e-6 Ohm  G_parasitic_PQ=1e-6 1/Ohm  Vmag0=12023.5058 V  Vang0=0 deg  Freq0=60 Hz  IL_specify=on  IL_priority=High  IL=[ 0 0 0 ] A  IL_nominal_specify=off  IL_nominal_value=1  IL_nominal_unit=A  VC_specify=on  VC_priority=High  VC=[ 0 0 0 ] V  VC_nominal_specify=off  VC_nominal_value=1  VC_nominal_unit=V
  A : PMIOPort  Side=Left
  B : PMIOPort  Port=2  Side=Left
  C : PMIOPort  Port=3  Side=Left
  connections:
  Electrical Reference/LConn1 -- Wye-Connected Load/RConn1
  Wye-Connected Load/LConn3 -- C/RConn1
  Wye-Connected Load/LConn1 -- A/RConn1
  Wye-Connected Load/LConn2 -- B/RConn1

== system IEEE33_TR_TEMPORAL_RECOGNIZABILITY_MASTER/Bus_6/Bus_6 ==
  Current and Voltage Sensor (Three-Phase) : ee_lib/Sensors & Transducers/Current and Voltage Sensor (Three-Phase)  port_option=ee.enum.threePhasePort.expanded  vMeasurementType=1  outputUnit=2  SRated=100000000 V*A  VRated=500000 V  I_specify=off  I_priority=None  I=[ 0 0 0 ] A  I_nominal_specify=off  I_nominal_value=1  I_nominal_unit=A  V_specify=off  V_priority=None  V=[ 0 0 0 ] V  V_nominal_specify=off  V_nominal_value=1  V_nominal_unit=V
  Igain : Gain  Gain=Three_PhaseV_IMeasuremen_class('phase-to-phase','yes','off','off','off',100000000,500000).objParamMappingDerived.NewDerivedParam.IG
  PS-Simulink Converter : nesl_utility/PS-Simulink Converter  PhysicalDomain=network_engine_domain  SubClassName=ps_output  LeftPortType=input  RightPortType=output  PseudoPeriodic=off  Frequencies=[]  VectorFormat=1-D array  Unit=1  AffineConversion=off
  PS-Simulink Converter1 : nesl_utility/PS-Simulink Converter  PhysicalDomain=network_engine_domain  SubClassName=ps_output  LeftPortType=input  RightPortType=output  PseudoPeriodic=off  Frequencies=[]  VectorFormat=1-D array  Unit=1  AffineConversion=off
  Vgain : Gain  Gain=Three_PhaseV_IMeasuremen_class('phase-to-phase','yes','off','off','off',100000000,500000).objParamMappingDerived.NewDerivedParam.VG
  A : PMIOPort  Side=Left
  B : PMIOPort  Port=2  Side=Left
  C : PMIOPort  Port=3  Side=Left
  a : PMIOPort  Port=4  Side=Right
  b : PMIOPort  Port=5  Side=Right
  c : PMIOPort  Port=6  Side=Right
  Vabc : Outport  VectorParamsAs1DForOutWhenUnconnected=off
  Iabc : Outport  Port=2  VectorParamsAs1DForOutWhenUnconnected=off
  wires:
  Igain/1 -> Iabc/1
  Vgain/1 -> Vabc/1
  PS-Simulink Converter1/1 -> Igain/1
  PS-Simulink Converter/1 -> Vgain/1
  connections:
  Current and Voltage Sensor (Three-Phase)/RConn1 -- PS-Simulink Converter/LConn1
  Current and Voltage Sensor (Three-Phase)/RConn2 -- PS-Simulink Converter1/LConn1
  Current and Voltage Sensor (Three-Phase)/RConn5 -- c/RConn1
  Current and Voltage Sensor (Three-Phase)/RConn4 -- b/RConn1
  Current and Voltage Sensor (Three-Phase)/RConn3 -- a/RConn1
  Current and Voltage Sensor (Three-Phase)/LConn3 -- C/RConn1
  Current and Voltage Sensor (Three-Phase)/LConn1 -- A/RConn1
  Current and Voltage Sensor (Three-Phase)/LConn2 -- B/RConn1

== system IEEE33_TR_TEMPORAL_RECOGNIZABILITY_MASTER/Bus_6/CB3-1 ==
  com : Inport
  Add : Sum
  Circuit Breaker : ee_lib/Switches & Breakers/Circuit Breaker (Three-Phase)  port_option=ee.enum.threePhasePort.expanded  control_port_option=ee.enum.controlport.ps  R_closed=0.01 Ohm  G_open=Three_PhaseBreaker_class('open',1000000,Inf,[0.0166666666666667 0.0833333333333333],'on').objParamMappingDerived.NewDerivedParam.G_open 1/Ohm  threshold=0.5 V  breaker_behavior=ee.enum.switches.breakerBehavior.zeroCrossingEnable  i_th=1e-8 A
  Data Type Conversion : DataTypeConversion  OutDataTypeStr=double  SaturateOnIntegerOverflow=off  RndMeth=Floor
  NOT : Logic  Operator=NOT  IconShape=distinctive  AllPortsSameDT=off  OutDataTypeStr=boolean
  Simulink-PS Converter : nesl_utility/Simulink-PS Converter  PhysicalDomain=network_engine_domain  SubClassName=ps_input  LeftPortType=input  RightPortType=output  PseudoPeriodic=off  Frequencies=[]  NoiseDistribution=none  NoiseParameters=[]  Unit=1  AffineConversion=off  FilteringAndDerivatives=provide  SimscapeFilterOrder=1  InputFilterTimeConstant=0.001  UdotUserProvided=0
  Step : Step  Time=1e-6  InitialValue=Three_PhaseBreaker_class('open',1000000,Inf,[0.0166666666666667 0.0833333333333333],'on').objParamMappingDerived.NewDerivedParam.StepInitialValue  FinalValue=0  SampleTime=0
  A : PMIOPort  Side=Left
  B : PMIOPort  Port=2  Side=Left
  C : PMIOPort  Port=3  Side=Left
  a : PMIOPort  Port=4  Side=Right
  b : PMIOPort  Port=5  Side=Right
  c : PMIOPort  Port=6  Side=Right
  wires:
  com/1 -> Add/1
  Add/1 -> NOT/1
  Step/1 -> Add/2
  Data Type Conversion/1 -> Simulink-PS Converter/1
  NOT/1 -> Data Type Conversion/1
  connections:
  Circuit Breaker/LConn1 -- Simulink-PS Converter/RConn1
  c/RConn1 -- Circuit Breaker/RConn3
  b/RConn1 -- Circuit Breaker/RConn2
  a/RConn1 -- Circuit Breaker/RConn1
  Circuit Breaker/LConn4 -- C/RConn1
  Circuit Breaker/LConn3 -- B/RConn1
  Circuit Breaker/LConn2 -- A/RConn1

== system IEEE33_TR_TEMPORAL_RECOGNIZABILITY_MASTER/Bus_6/CB3-2 ==
  com : Inport
  Add : Sum
  Circuit Breaker : ee_lib/Switches & Breakers/Circuit Breaker (Three-Phase)  port_option=ee.enum.threePhasePort.expanded  control_port_option=ee.enum.controlport.ps  R_closed=0.01 Ohm  G_open=Three_PhaseBreaker_class('open',1000000,Inf,[0.0166666666666667 0.0833333333333333],'on').objParamMappingDerived.NewDerivedParam.G_open 1/Ohm  threshold=0.5 V  breaker_behavior=ee.enum.switches.breakerBehavior.zeroCrossingEnable  i_th=1e-8 A
  Data Type Conversion : DataTypeConversion  OutDataTypeStr=double  SaturateOnIntegerOverflow=off  RndMeth=Floor
  NOT : Logic  Operator=NOT  IconShape=distinctive  AllPortsSameDT=off  OutDataTypeStr=boolean
  Simulink-PS Converter : nesl_utility/Simulink-PS Converter  PhysicalDomain=network_engine_domain  SubClassName=ps_input  LeftPortType=input  RightPortType=output  PseudoPeriodic=off  Frequencies=[]  NoiseDistribution=none  NoiseParameters=[]  Unit=1  AffineConversion=off  FilteringAndDerivatives=provide  SimscapeFilterOrder=1  InputFilterTimeConstant=0.001  UdotUserProvided=0
  Step : Step  Time=1e-6  InitialValue=Three_PhaseBreaker_class('open',1000000,Inf,[0.0166666666666667 0.0833333333333333],'on').objParamMappingDerived.NewDerivedParam.StepInitialValue  FinalValue=0  SampleTime=0
  A : PMIOPort  Side=Left
  B : PMIOPort  Port=2  Side=Left
  C : PMIOPort  Port=3  Side=Left
  a : PMIOPort  Port=4  Side=Right
  b : PMIOPort  Port=5  Side=Right
  c : PMIOPort  Port=6  Side=Right
  wires:
  com/1 -> Add/1
  Add/1 -> NOT/1
  Step/1 -> Add/2
  Data Type Conversion/1 -> Simulink-PS Converter/1
  NOT/1 -> Data Type Conversion/1
  connections:
  Circuit Breaker/LConn1 -- Simulink-PS Converter/RConn1
  c/RConn1 -- Circuit Breaker/RConn3
  b/RConn1 -- Circuit Breaker/RConn2
  a/RConn1 -- Circuit Breaker/RConn1
  Circuit Breaker/LConn4 -- C/RConn1
  Circuit Breaker/LConn3 -- B/RConn1
  Circuit Breaker/LConn2 -- A/RConn1

== system IEEE33_TR_TEMPORAL_RECOGNIZABILITY_MASTER/Bus_6/VI Recorder9 ==
  Vrec : Inport
  Irec : Inport  Port=2
  tag scope: I5to6=global, V5to6=global
  wires:
  Vrec/1 -> [V5to6]
  Irec/1 -> [I5to6]

== system IEEE33_TR_TEMPORAL_RECOGNIZABILITY_MASTER/Bus_7/Bus Load 7 ==
  Electrical Reference : fl_lib/Electrical/Electrical Elements/Electrical Reference
  Wye-Connected Load : ee_lib/Passive/RLC Assemblies/Wye-Connected Load  port_option=ee.enum.threePhasePort.expanded  parameterization=2  component_structure=4  component_structure_PQ=4  R=1 Ohm  L=0.001 H  C=1e-6 F  VRated=11979.4364 V  FRated=60 Hz  P=200000 W  Qpos=100000 V*A  Qneg=Three_PhaseSeriesRLCLoad_class(0).objParamMappingDerived.NewDerivedParam.Qneg V*A  R_parasitic=1e-6 Ohm  G_parasitic=1e-6 1/Ohm  R_parasitic_PQ=1e-6 Ohm  G_parasitic_PQ=1e-6 1/Ohm  Vmag0=11979.4364 V  Vang0=0 deg  Freq0=60 Hz  IL_specify=on  IL_priority=High  IL=[ 0 0 0 ] A  IL_nominal_specify=off  IL_nominal_value=1  IL_nominal_unit=A  VC_specify=on  VC_priority=High  VC=[ 0 0 0 ] V  VC_nominal_specify=off  VC_nominal_value=1  VC_nominal_unit=V
  A : PMIOPort  Side=Left
  B : PMIOPort  Port=2  Side=Left
  C : PMIOPort  Port=3  Side=Left
  connections:
  Electrical Reference/LConn1 -- Wye-Connected Load/RConn1
  Wye-Connected Load/LConn3 -- C/RConn1
  Wye-Connected Load/LConn1 -- A/RConn1
  Wye-Connected Load/LConn2 -- B/RConn1

== system IEEE33_TR_TEMPORAL_RECOGNIZABILITY_MASTER/Bus_7/Bus_7 ==
  Current and Voltage Sensor (Three-Phase) : ee_lib/Sensors & Transducers/Current and Voltage Sensor (Three-Phase)  port_option=ee.enum.threePhasePort.expanded  vMeasurementType=1  outputUnit=2  SRated=100000000 V*A  VRated=500000 V  I_specify=off  I_priority=None  I=[ 0 0 0 ] A  I_nominal_specify=off  I_nominal_value=1  I_nominal_unit=A  V_specify=off  V_priority=None  V=[ 0 0 0 ] V  V_nominal_specify=off  V_nominal_value=1  V_nominal_unit=V
  Igain : Gain  Gain=Three_PhaseV_IMeasuremen_class('phase-to-phase','yes','off','off','off',100000000,500000).objParamMappingDerived.NewDerivedParam.IG
  PS-Simulink Converter : nesl_utility/PS-Simulink Converter  PhysicalDomain=network_engine_domain  SubClassName=ps_output  LeftPortType=input  RightPortType=output  PseudoPeriodic=off  Frequencies=[]  VectorFormat=1-D array  Unit=1  AffineConversion=off
  PS-Simulink Converter1 : nesl_utility/PS-Simulink Converter  PhysicalDomain=network_engine_domain  SubClassName=ps_output  LeftPortType=input  RightPortType=output  PseudoPeriodic=off  Frequencies=[]  VectorFormat=1-D array  Unit=1  AffineConversion=off
  Vgain : Gain  Gain=Three_PhaseV_IMeasuremen_class('phase-to-phase','yes','off','off','off',100000000,500000).objParamMappingDerived.NewDerivedParam.VG
  A : PMIOPort  Side=Left
  B : PMIOPort  Port=2  Side=Left
  C : PMIOPort  Port=3  Side=Left
  a : PMIOPort  Port=4  Side=Right
  b : PMIOPort  Port=5  Side=Right
  c : PMIOPort  Port=6  Side=Right
  Vabc : Outport  VectorParamsAs1DForOutWhenUnconnected=off
  Iabc : Outport  Port=2  VectorParamsAs1DForOutWhenUnconnected=off
  wires:
  Igain/1 -> Iabc/1
  Vgain/1 -> Vabc/1
  PS-Simulink Converter1/1 -> Igain/1
  PS-Simulink Converter/1 -> Vgain/1
  connections:
  Current and Voltage Sensor (Three-Phase)/RConn1 -- PS-Simulink Converter/LConn1
  Current and Voltage Sensor (Three-Phase)/RConn2 -- PS-Simulink Converter1/LConn1
  Current and Voltage Sensor (Three-Phase)/RConn5 -- c/RConn1
  Current and Voltage Sensor (Three-Phase)/RConn4 -- b/RConn1
  Current and Voltage Sensor (Three-Phase)/RConn3 -- a/RConn1
  Current and Voltage Sensor (Three-Phase)/LConn3 -- C/RConn1
  Current and Voltage Sensor (Three-Phase)/LConn1 -- A/RConn1
  Current and Voltage Sensor (Three-Phase)/LConn2 -- B/RConn1

== system IEEE33_TR_TEMPORAL_RECOGNIZABILITY_MASTER/Bus_7/CB3-2 ==
  com : Inport
  Add : Sum
  Circuit Breaker : ee_lib/Switches & Breakers/Circuit Breaker (Three-Phase)  port_option=ee.enum.threePhasePort.expanded  control_port_option=ee.enum.controlport.ps  R_closed=0.01 Ohm  G_open=Three_PhaseBreaker_class('open',1000000,Inf,[0.0166666666666667 0.0833333333333333],'on').objParamMappingDerived.NewDerivedParam.G_open 1/Ohm  threshold=0.5 V  breaker_behavior=ee.enum.switches.breakerBehavior.zeroCrossingEnable  i_th=1e-8 A
  Data Type Conversion : DataTypeConversion  OutDataTypeStr=double  SaturateOnIntegerOverflow=off  RndMeth=Floor
  NOT : Logic  Operator=NOT  IconShape=distinctive  AllPortsSameDT=off  OutDataTypeStr=boolean
  Simulink-PS Converter : nesl_utility/Simulink-PS Converter  PhysicalDomain=network_engine_domain  SubClassName=ps_input  LeftPortType=input  RightPortType=output  PseudoPeriodic=off  Frequencies=[]  NoiseDistribution=none  NoiseParameters=[]  Unit=1  AffineConversion=off  FilteringAndDerivatives=provide  SimscapeFilterOrder=1  InputFilterTimeConstant=0.001  UdotUserProvided=0
  Step : Step  Time=1e-6  InitialValue=Three_PhaseBreaker_class('open',1000000,Inf,[0.0166666666666667 0.0833333333333333],'on').objParamMappingDerived.NewDerivedParam.StepInitialValue  FinalValue=0  SampleTime=0
  A : PMIOPort  Side=Left
  B : PMIOPort  Port=2  Side=Left
  C : PMIOPort  Port=3  Side=Left
  a : PMIOPort  Port=4  Side=Right
  b : PMIOPort  Port=5  Side=Right
  c : PMIOPort  Port=6  Side=Right
  wires:
  com/1 -> Add/1
  Add/1 -> NOT/1
  Step/1 -> Add/2
  Data Type Conversion/1 -> Simulink-PS Converter/1
  NOT/1 -> Data Type Conversion/1
  connections:
  Circuit Breaker/LConn1 -- Simulink-PS Converter/RConn1
  c/RConn1 -- Circuit Breaker/RConn3
  b/RConn1 -- Circuit Breaker/RConn2
  a/RConn1 -- Circuit Breaker/RConn1
  Circuit Breaker/LConn4 -- C/RConn1
  Circuit Breaker/LConn3 -- B/RConn1
  Circuit Breaker/LConn2 -- A/RConn1
